simulink model "telescopio"  (R2025b)
settings: Solver=VariableStepAuto  StartTime=0.0  StopTime=15  RelTol=1e-3  AbsTol=1e-3
undefined symbols (not defined in the file): X, Y, Z
libraries: fl_lib x22, sm_lib x17, nesl_utility x17, ee_lib x6, slpidlib x3, simulink x3, sdl_lib x2
settings Model: Creator=kl247  LastModifiedBy=kl247
settings SolverCC: AutoScaleAbsTol=off  ZeroCrossAlgorithm=Adaptive  AlgebraicLoopSolver=TrustRegion  MaxZcPerStep=1.0
settings DebuggingCC: IgnoredZcDiagnostic=none  UnconnectedInputMsg=warning  UnconnectedOutputMsg=warning  UnconnectedLineMsg=warning  SymbolicDimsDataTypeCodeGenerationDiagnostic=none
settings ModelReferenceCC: EnableRefExpFcnMdlSchedulingChecks=on
settings SFSimCC: CustomCodeUndefinedFunction=UseInterfaceOnly
settings RTWCC: GPUComputeCapability=3.5  DLArmComputeVersion=19.05
settings SimscapeCC: SimscapeLogType=all  SimscapeLogSimulationStatistics=on  SimscapeLogDataHistory=10000.0

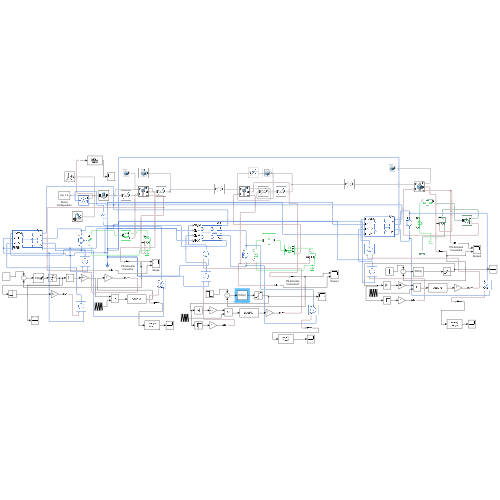
[thumbnail: Simulink's stored preview of the top-level diagram]
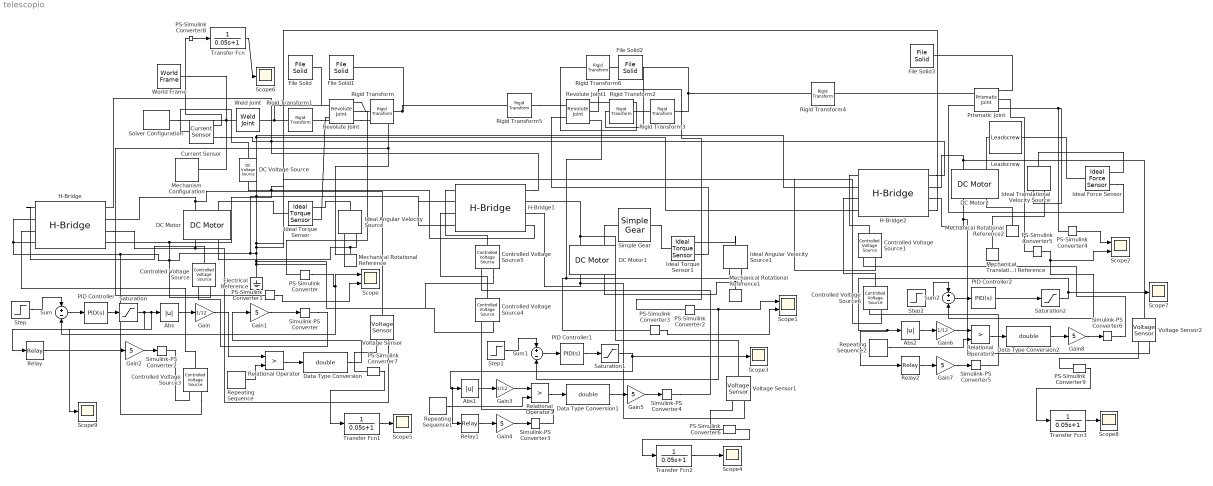
== system telescopio ==
  Abs : Abs  ZeroCross=off  SaturateOnIntegerOverflow=off
  Abs1 : Abs  ZeroCross=off  SaturateOnIntegerOverflow=off
  Abs2 : Abs  ZeroCross=off  SaturateOnIntegerOverflow=off
  Controlled Voltage Source{,1,3..6} (6 alike) : fl_lib/Electrical/Electrical Sources/Controlled Voltage Source
  Current Sensor : fl_lib/Electrical/Electrical Sensors/Current Sensor
  DC Motor : ee_lib/Electromechanical/Brushed Motors/DC Motor  field_option=ee.enum.field_option.pm  Rf=100 Ohm  Lf=1 H  Laf=0.15 H  If0=0 A  parameterization=ee.enum.dcparam_option.circuit_param  Ra=3.9 Ohm  La=12e-6 H  emf_or_torque=ee.enum.emf_or_torque.kv  Kv=0.072e-3 V/rpm  Ki=6.876e-4 N*m/A  T_stall=0.24e-3 N*m  w_max=19100 rpm  w_rated=15000 rpm  P_rated=0.08 W  V_rated=1.5 V  lam_param=ee.enum.lam_param.damping  i_noload=0 A  V_i_noload=1.5 V  J=0.01 cm^2*g  lam=0 N*m*s/rad  speed0=0 rpm  alpha=3.93e-3 1/K  Tmeas=25 degC  thermal_mass=100 J/K  initial_temperature=25 degC
  DC Motor1 : ee_lib/Electromechanical/Brushed Motors/DC Motor  field_option=ee.enum.field_option.pm  Rf=100 Ohm  Lf=1 H  Laf=0.15 H  If0=0 A  parameterization=ee.enum.dcparam_option.circuit_param  Ra=3.9 Ohm  La=12e-6 H  emf_or_torque=ee.enum.emf_or_torque.kv  Kv=0.072e-3 V/rpm  Ki=6.876e-4 N*m/A  T_stall=0.24e-3 N*m  w_max=19100 rpm  w_rated=15000 rpm  P_rated=0.08 W  V_rated=1.5 V  lam_param=ee.enum.lam_param.damping  i_noload=0 A  V_i_noload=1.5 V  J=0.01 cm^2*g  lam=0 N*m*s/rad  speed0=0 rpm  alpha=3.93e-3 1/K  Tmeas=25 degC  thermal_mass=100 J/K  initial_temperature=25 degC
  DC Motor2 : ee_lib/Electromechanical/Brushed Motors/DC Motor  field_option=ee.enum.field_option.pm  Rf=100 Ohm  Lf=1 H  Laf=0.15 H  If0=0 A  parameterization=ee.enum.dcparam_option.circuit_param  Ra=3.9 Ohm  La=12e-6 H  emf_or_torque=ee.enum.emf_or_torque.kv  Kv=0.072e-3 V/rpm  Ki=6.876e-4 N*m/A  T_stall=0.24e-3 N*m  w_max=19100 rpm  w_rated=15000 rpm  P_rated=0.08 W  V_rated=1.5 V  lam_param=ee.enum.lam_param.damping  i_noload=0 A  V_i_noload=1.5 V  J=0.01 cm^2*g  lam=0 N*m*s/rad  speed0=0 rpm  alpha=3.93e-3 1/K  Tmeas=25 degC  thermal_mass=100 J/K  initial_temperature=25 degC
  DC Voltage Source : fl_lib/Electrical/Electrical Sources/DC Voltage Source  v0=12 V
  Data Type Conversion : DataTypeConversion  OutDataTypeStr=double  SaturateOnIntegerOverflow=off  RndMeth=Floor
  Data Type Conversion1 : DataTypeConversion  OutDataTypeStr=double  SaturateOnIntegerOverflow=off  RndMeth=Floor
  Data Type Conversion2 : DataTypeConversion  OutDataTypeStr=double  SaturateOnIntegerOverflow=off  RndMeth=Floor
  Electrical Reference : fl_lib/Electrical/Electrical Elements/Electrical Reference
  File Solid : sm_lib/Body Elements/File Solid  ExtGeomFileName=C:\Users\kl247\OneDrive\Desktop\base_telescopio1.STEP  UnitType=FromFile  ExtGeomFileUnits=m  StepReaderType=HEX  ExportConvexHullGeometry=off  InertiaType=CalculateFromGeometry  BasedOnType=Density  Density=1200  DensityUnits=kg/m^3  Mass=1  MassUnits=kg  CenterOfMass=[0 0 0]  CenterOfMassUnits=m  MomentsOfInertia=[1 1 1]  MomentsOfInertiaUnits=kg*m^2  ProductsOfInertia=[0 0 0]  ProductsOfInertiaUnits=kg*m^2  GraphicType=FromGeometry  MarkerShape=Sphere  MarkerSize=10  GraphicVisPropType=SimpleVisualProperties  GraphicDiffuseColor=[0.5 0.5 0.5]  GraphicOpacity=1  GraphicSpecularColor=[0.5 0.5 0.5 1.0]  GraphicAmbientColor=[0.15 0.15 0.15 1.0]  GraphicEmissiveColor=[0.0 0.0 0.0 1.0]  GraphicShininess=75  DoExposeReferenceFrame=on  SerializedFrames=<Frames/>
  File Solid1 : sm_lib/Body Elements/File Solid  ExtGeomFileName=C:\Users\kl247\OneDrive\Desktop\soporte.STEP1.STEP  UnitType=FromFile  ExtGeomFileUnits=m  StepReaderType=HEX  ExportConvexHullGeometry=off  InertiaType=CalculateFromGeometry  BasedOnType=Density  Density=1200  DensityUnits=kg/m^3  Mass=1  MassUnits=kg  CenterOfMass=[0 0 0]  CenterOfMassUnits=m  MomentsOfInertia=[1 1 1]  MomentsOfInertiaUnits=kg*m^2  ProductsOfInertia=[0 0 0]  ProductsOfInertiaUnits=kg*m^2  GraphicType=FromGeometry  MarkerShape=Sphere  MarkerSize=10  GraphicVisPropType=SimpleVisualProperties  GraphicDiffuseColor=[0.5 0.5 0.5]  GraphicOpacity=1  GraphicSpecularColor=[0.5 0.5 0.5 1.0]  GraphicAmbientColor=[0.15 0.15 0.15 1.0]  GraphicEmissiveColor=[0.0 0.0 0.0 1.0]  GraphicShininess=75  DoExposeReferenceFrame=on  SerializedFrames=<Frames/>
  File Solid2 : sm_lib/Body Elements/File Solid  ExtGeomFileName=C:\Users\kl247\OneDrive\Desktop\tubo_exterior.STEP  UnitType=FromFile  ExtGeomFileUnits=m  StepReaderType=HEX  ExportConvexHullGeometry=off  InertiaType=CalculateFromGeometry  BasedOnType=Density  Density=300  DensityUnits=kg/m^3  Mass=1  MassUnits=kg  CenterOfMass=[0 0 0]  CenterOfMassUnits=m  MomentsOfInertia=[1 1 1]  MomentsOfInertiaUnits=kg*m^2  ProductsOfInertia=[0 0 0]  ProductsOfInertiaUnits=kg*m^2  GraphicType=FromGeometry  MarkerShape=Sphere  MarkerSize=10  GraphicVisPropType=SimpleVisualProperties  GraphicDiffuseColor=[0.5 0.5 0.5]  GraphicOpacity=1  GraphicSpecularColor=[0.5 0.5 0.5 1.0]  GraphicAmbientColor=[0.15 0.15 0.15 1.0]  GraphicEmissiveColor=[0.0 0.0 0.0 1.0]  GraphicShininess=75  DoExposeReferenceFrame=on  SerializedFrames=<Frames/>
  File Solid3 : sm_lib/Body Elements/File Solid  ExtGeomFileName=C:\Users\kl247\OneDrive\Desktop\tubo_interior.STEP  UnitType=FromFile  ExtGeomFileUnits=m  StepReaderType=HEX  ExportConvexHullGeometry=off  InertiaType=CalculateFromGeometry  BasedOnType=Density  Density=300  DensityUnits=kg/m^3  Mass=1  MassUnits=kg  CenterOfMass=[0 0 0]  CenterOfMassUnits=m  MomentsOfInertia=[1 1 1]  MomentsOfInertiaUnits=kg*m^2  ProductsOfInertia=[0 0 0]  ProductsOfInertiaUnits=kg*m^2  GraphicType=FromGeometry  MarkerShape=Sphere  MarkerSize=10  GraphicVisPropType=SimpleVisualProperties  GraphicDiffuseColor=[0.5 0.5 0.5]  GraphicOpacity=1  GraphicSpecularColor=[0.5 0.5 0.5 1.0]  GraphicAmbientColor=[0.15 0.15 0.15 1.0]  GraphicEmissiveColor=[0.0 0.0 0.0 1.0]  GraphicShininess=75  DoExposeReferenceFrame=on  SerializedFrames=<Frames/>
  Gain : Gain  Gain=1/12
  Gain{1..2,4..5,7..8} (6 alike) : Gain  Gain=5
  Gain3 : Gain  Gain=1/12
  Gain6 : Gain  Gain=1/12
  H-Bridge : ee_lib/Semiconductors & Converters/Converters/H-Bridge  supply_ports=ee.enum.supply_ports.showsupply  pwm_or_av=ee.enum.pwm_or_av.pwm  regenerative_braking_mode=ee.enum.converters.regenerative_braking_mode.depends_on_rev  discontinuous=ee.enum.current_profile.continuous  freewheeling_mode=ee.enum.converters.freewheeling_mode.one_switch_one_diode  Rload=10 Ohm  Lload=1e-5 H  F=10 kHz  Venable=2.5 V  Vmax=5.0 V  Vreverse=2.5 V  Vbrake=2.5 V  Vm=12 V  Ron=0.1 Ohm  Don=0.05 Ohm  Goff=1e-6 S  Tmeas=298.15 K  Ron2=0.1 Ohm  Don2=0.05 Ohm  Tmeas2=398.15 K  thermal_mass=100 J/K  initial_temperature=298.15 K
      settings: InternalSimscapePortConfiguration="{\"Bottom\":[],\"Left\":[{\"id\":\"ENA\",\"label\":\"PWM\",\"type\":\"foundation.electrical.electrical\"},{\"id\":\"REF\",\"label\":\"REF\",\"type\":\"foundation.electrical.electrical\"},{\"id\":\"REV\",\"label\":\"REV\",\"type\":\"foundation.electrical.electrical\"},{\"id\":\"BRK\",\"label\":\"BRK\",\"type\":\"foundation.electrical.electrical\"}],\"Right\":[{\"id\":\"p1\",\"label\":\"V+\",\"type\":\"foundation.electrical.electrical\"},{\"id\":\"p2\",\"label\":\"+\",\"type\":\"foundation.electrical.electrical\"},{\"id\":\"n2\",\"label\":\"-\",\"type\":\"foundation.electrical.electrical\"},{\"id\":\"n1\",\"label\":\"V-\",\"type\":\"foundation.electrical.electrical\"}],\"Top\":[]}"
  H-Bridge1 : ee_lib/Semiconductors & Converters/Converters/H-Bridge  supply_ports=ee.enum.supply_ports.showsupply  pwm_or_av=ee.enum.pwm_or_av.pwm  regenerative_braking_mode=ee.enum.converters.regenerative_braking_mode.depends_on_rev  discontinuous=ee.enum.current_profile.continuous  freewheeling_mode=ee.enum.converters.freewheeling_mode.one_switch_one_diode  Rload=10 Ohm  Lload=1e-5 H  F=10 kHz  Venable=2.5 V  Vmax=5.0 V  Vreverse=2.5 V  Vbrake=2.5 V  Vm=12 V  Ron=0.1 Ohm  Don=0.05 Ohm  Goff=1e-6 S  Tmeas=298.15 K  Ron2=0.1 Ohm  Don2=0.05 Ohm  Tmeas2=398.15 K  thermal_mass=100 J/K  initial_temperature=298.15 K
      settings: InternalSimscapePortConfiguration="{\"Bottom\":[],\"Left\":[{\"id\":\"ENA\",\"label\":\"PWM\",\"type\":\"foundation.electrical.electrical\"},{\"id\":\"REF\",\"label\":\"REF\",\"type\":\"foundation.electrical.electrical\"},{\"id\":\"REV\",\"label\":\"REV\",\"type\":\"foundation.electrical.electrical\"},{\"id\":\"BRK\",\"label\":\"BRK\",\"type\":\"foundation.electrical.electrical\"}],\"Right\":[{\"id\":\"p1\",\"label\":\"V+\",\"type\":\"foundation.electrical.electrical\"},{\"id\":\"p2\",\"label\":\"+\",\"type\":\"foundation.electrical.electrical\"},{\"id\":\"n2\",\"label\":\"-\",\"type\":\"foundation.electrical.electrical\"},{\"id\":\"n1\",\"label\":\"V-\",\"type\":\"foundation.electrical.electrical\"}],\"Top\":[]}"
  H-Bridge2 : ee_lib/Semiconductors & Converters/Converters/H-Bridge  supply_ports=ee.enum.supply_ports.showsupply  pwm_or_av=ee.enum.pwm_or_av.pwm  regenerative_braking_mode=ee.enum.converters.regenerative_braking_mode.depends_on_rev  discontinuous=ee.enum.current_profile.continuous  freewheeling_mode=ee.enum.converters.freewheeling_mode.one_switch_one_diode  Rload=10 Ohm  Lload=1e-5 H  F=10 kHz  Venable=2.5 V  Vmax=5.0 V  Vreverse=2.5 V  Vbrake=2.5 V  Vm=12 V  Ron=0.1 Ohm  Don=0.05 Ohm  Goff=1e-6 S  Tmeas=298.15 K  Ron2=0.1 Ohm  Don2=0.05 Ohm  Tmeas2=398.15 K  thermal_mass=100 J/K  initial_temperature=298.15 K
      settings: InternalSimscapePortConfiguration="{\"Bottom\":[],\"Left\":[{\"id\":\"ENA\",\"label\":\"PWM\",\"type\":\"foundation.electrical.electrical\"},{\"id\":\"REF\",\"label\":\"REF\",\"type\":\"foundation.electrical.electrical\"},{\"id\":\"REV\",\"label\":\"REV\",\"type\":\"foundation.electrical.electrical\"},{\"id\":\"BRK\",\"label\":\"BRK\",\"type\":\"foundation.electrical.electrical\"}],\"Right\":[{\"id\":\"p1\",\"label\":\"V+\",\"type\":\"foundation.electrical.electrical\"},{\"id\":\"p2\",\"label\":\"+\",\"type\":\"foundation.electrical.electrical\"},{\"id\":\"n2\",\"label\":\"-\",\"type\":\"foundation.electrical.electrical\"},{\"id\":\"n1\",\"label\":\"V-\",\"type\":\"foundation.electrical.electrical\"}],\"Top\":[]}"
  Ideal Angular Velocity Source : fl_lib/Mechanical/Mechanical Sources/Ideal Angular Velocity Source
  Ideal Angular Velocity Source1 : fl_lib/Mechanical/Mechanical Sources/Ideal Angular Velocity Source
  Ideal Force Sensor : fl_lib/Mechanical/Mechanical Sensors/Ideal Force Sensor
  Ideal Torque Sensor : fl_lib/Mechanical/Mechanical Sensors/Ideal Torque Sensor
  Ideal Torque Sensor1 : fl_lib/Mechanical/Mechanical Sensors/Ideal Torque Sensor
  Ideal Translational Velocity Source : fl_lib/Mechanical/Mechanical Sources/Ideal Translational Velocity Source
  Leadscrew : sdl_lib/Gears/Rotational- Translational/Leadscrew  Lead=0.015 m  helix_type=sdl.enum.handedness.right  friction_model=sdl.enum.gear_friction.none  friction_parameterization=sdl.enum.frictionParameterization.geometry  lambda=15 deg  alpha=14.5 deg  fr_coeff=0.08  eff_sn=0.75  eff_ns=0.45  temperature_TLU=[280, 300, 320] K  efficiency_sn_TLU=[.75, .65, .6]  efficiency_ns_TLU=[.5, .45, .4]  pwr_thr=0.001 W  mu_visc=0 N*m*s/rad  thermal_mass=50 J/K  temperature_specify=off  temperature_priority=High  temperature=300 K  temperature_nominal_specify=off  temperature_nominal_value=1  temperature_nominal_unit=K
      settings: InternalSimscapePortConfiguration="{\"Bottom\":[],\"Left\":[{\"id\":\"S\",\"label\":\"S\",\"type\":\"foundation.mechanical.rotational.rotational\"}],\"Right\":[{\"id\":\"N\",\"label\":\"N\",\"type\":\"foundation.mechanical.translational.translational\"}],\"Top\":[]}"
  Mechanical Rotational Reference : fl_lib/Mechanical/Rotational Elements/Mechanical Rotational Reference
  Mechanical Rotational Reference1 : fl_lib/Mechanical/Rotational Elements/Mechanical Rotational Reference
  Mechanical Rotational Reference2 : fl_lib/Mechanical/Rotational Elements/Mechanical Rotational Reference
  Mechanical Translational Reference : fl_lib/Mechanical/Translational Elements/Mechanical Translational Reference
  Mechanism Configuration : sm_lib/Utilities/Mechanism Configuration  UniformGravity=Constant  GravityVector=[0 0 -9.80665]  GravityVectorUnits=m/s^2  LinearizationDelta=0.001  JointModeTransitionNonlinearIterations=2
  PID Controller : slpidlib/PID Controller  Controller=PID  Form=Parallel  TimeDomain=Continuous-time  UseExternalTs=off  SampleTime=-1  IntegratorMethod=Forward Euler  FilterMethod=Forward Euler  ControllerParametersSource=internal  P=3  I=0  UseKiTs=off  D=10  UseExternalDerivativeSource=off  N=100  UseFilter=on  TunerSelectOption=Transfer Function Based (PID Tuner App)  InitialConditionSource=internal  InitialConditionForIntegrator=0  InitialConditionForFilter=0  DifferentiatorICPrevScaledInput=0  ExternalReset=none  TrackingMode=off  Kt=1  LimitOutput=on  SatLimitsSource=internal  UpperSaturationLimit=12  LowerSaturationLimit=-12  LinearizeAsGain=on  AntiWindupMode=none  Kb=1  LimitIntegrator=off  UpperIntegratorSaturationLimit=inf  LowerIntegratorSaturationLimit=-inf  POutMin=[]  POutMax=[]  IOutMin=[]  IOutMax=[]  DOutMin=[]  DOutMax=[]  NOutMin=[]  NOutMax=[]  SumOutMin=[]  SumOutMax=[]  SaturationOutMin=[]  SaturationOutMax=[]  PParamMin=[]  PParamMax=[]  IParamMin=[]  IParamMax=[]  DParamMin=[]  DParamMax=[]  NParamMin=[]  NParamMax=[]  KbParamMin=[]  KbParamMax=[]  KtParamMin=[]  KtParamMax=[]  KbOutMin=[]  KbOutMax=[]  KtOutMin=[]  KtOutMax=[]  IntegratorOutMin=[]  IntegratorOutMax=[]  FilterOutMin=[]  FilterOutMax=[]  SumI1OutMin=[]  SumI1OutMax=[]  SumI2OutMin=[]  SumI2OutMax=[]  SumI3OutMin=[]  SumI3OutMax=[]  SumI4OutMin=[]  SumI4OutMax=[]  SumDOutMin=[]  SumDOutMax=[]  DifferentiatorOutMin=[]  DifferentiatorOutMax=[]  FilterDiffOutCoefMin=[]  FilterDiffOutCoefMax=[]  ReciprocalOutMin=[]  ReciprocalOutMax=[]  SumDenOutMin=[]  SumDenOutMax=[]  SumNumOutMin=[]  SumNumOutMax=[]  DivideOutMin=[]  DivideOutMax=[]  UdiffTsProdOutMin=[]  UdiffTsProdOutMax=[]  NTsProdOutMin=[]  NTsProdOutMax=[]  UintegralTsProdOutMin=[]  UintegralTsProdOutMax=[]  UngainTsProdOutMin=[]  UngainTsProdOutMax=[]  ClampingZeroOutDataTypeStr=Inherit: Inherit via back propagation  ClampingZeroOutMin=[]  ClampingZeroOutMax=[]  FilterDenConstantOutDataTypeStr=Inherit: Inherit via back propagation  FilterDenConstantOutMin=[]  FilterDenConstantOutMax=[]  PCopyOutDataTypeStr=Inherit: Inherit via back propagation  PCopyOutMin=[]  PCopyOutMax=[]  NCopyOutDataTypeStr=Inherit: Inherit via back propagation  NCopyOutMin=[]  NCopyOutMax=[]  IntegratorContinuousStateAttributes=''  IntegratorStateMustResolveToSignalObject=off  IntegratorRTWStateStorageClass=Auto  FilterContinuousStateAttributes=''  FilterStateMustResolveToSignalObject=off  FilterRTWStateStorageClass=Auto  ParallelPVariant=InternalParameters  IdealPVariant=Disabled  IVariant=InternalParameters  DVariant=InternalParameters  IntegratorVariant=Continuous  SatVariant=Enabled  AWVariant=Passthrough  PCopyVariant=Disabled  TRVariant=Disabled  FdbkBlocksVariant=Forward  IdealPFdbkVariant=Disabled  SatFdbkVariant=Disabled  DerivativeFilterVariant=ContFilter  NVariant=InternalParameters  NCopyVariant=Disabled  FilterICVariant=InternalICsFilter  IntegratorICVariant=InternalICs  ExternalResetVariant=Disabled  TRSumVariant=Passthrough  SumFdbkVariant=Disabled  SumVariant=Sum_PID  TsampFilterVariant=InternalTs  TsampNgainVariant=Passthrough  TsampIntegralVariant=Disabled_SignalSpec  ExternalSaturationOutDataTypeStr=Inherit: Same as second input  DerivativeSourceVariant=ErrorSignal  PreIntVariant=InternalPreInt
  PID Controller1 : slpidlib/PID Controller  Controller=PID  Form=Parallel  TimeDomain=Continuous-time  UseExternalTs=off  SampleTime=-1  IntegratorMethod=Forward Euler  FilterMethod=Forward Euler  ControllerParametersSource=internal  P=30  I=2  UseKiTs=off  D=10  UseExternalDerivativeSource=off  N=100  UseFilter=on  TunerSelectOption=Transfer Function Based (PID Tuner App)  InitialConditionSource=internal  InitialConditionForIntegrator=0  InitialConditionForFilter=0  DifferentiatorICPrevScaledInput=0  ExternalReset=none  TrackingMode=off  Kt=1  LimitOutput=off  SatLimitsSource=internal  UpperSaturationLimit=inf  LowerSaturationLimit=-inf  LinearizeAsGain=on  AntiWindupMode=none  Kb=1  LimitIntegrator=off  UpperIntegratorSaturationLimit=inf  LowerIntegratorSaturationLimit=-inf  POutMin=[]  POutMax=[]  IOutMin=[]  IOutMax=[]  DOutMin=[]  DOutMax=[]  NOutMin=[]  NOutMax=[]  SumOutMin=[]  SumOutMax=[]  SaturationOutMin=[]  SaturationOutMax=[]  PParamMin=[]  PParamMax=[]  IParamMin=[]  IParamMax=[]  DParamMin=[]  DParamMax=[]  NParamMin=[]  NParamMax=[]  KbParamMin=[]  KbParamMax=[]  KtParamMin=[]  KtParamMax=[]  KbOutMin=[]  KbOutMax=[]  KtOutMin=[]  KtOutMax=[]  IntegratorOutMin=[]  IntegratorOutMax=[]  FilterOutMin=[]  FilterOutMax=[]  SumI1OutMin=[]  SumI1OutMax=[]  SumI2OutMin=[]  SumI2OutMax=[]  SumI3OutMin=[]  SumI3OutMax=[]  SumI4OutMin=[]  SumI4OutMax=[]  SumDOutMin=[]  SumDOutMax=[]  DifferentiatorOutMin=[]  DifferentiatorOutMax=[]  FilterDiffOutCoefMin=[]  FilterDiffOutCoefMax=[]  ReciprocalOutMin=[]  ReciprocalOutMax=[]  SumDenOutMin=[]  SumDenOutMax=[]  SumNumOutMin=[]  SumNumOutMax=[]  DivideOutMin=[]  DivideOutMax=[]  UdiffTsProdOutMin=[]  UdiffTsProdOutMax=[]  NTsProdOutMin=[]  NTsProdOutMax=[]  UintegralTsProdOutMin=[]  UintegralTsProdOutMax=[]  UngainTsProdOutMin=[]  UngainTsProdOutMax=[]  ClampingZeroOutDataTypeStr=Inherit: Inherit via back propagation  ClampingZeroOutMin=[]  ClampingZeroOutMax=[]  FilterDenConstantOutDataTypeStr=Inherit: Inherit via back propagation  FilterDenConstantOutMin=[]  FilterDenConstantOutMax=[]  PCopyOutDataTypeStr=Inherit: Inherit via back propagation  PCopyOutMin=[]  PCopyOutMax=[]  NCopyOutDataTypeStr=Inherit: Inherit via back propagation  NCopyOutMin=[]  NCopyOutMax=[]  IntegratorContinuousStateAttributes=''  IntegratorStateMustResolveToSignalObject=off  IntegratorRTWStateStorageClass=Auto  FilterContinuousStateAttributes=''  FilterStateMustResolveToSignalObject=off  FilterRTWStateStorageClass=Auto  ParallelPVariant=InternalParameters  IdealPVariant=Disabled  IVariant=InternalParameters  DVariant=InternalParameters  IntegratorVariant=Continuous  SatVariant=Disabled  AWVariant=Passthrough  PCopyVariant=Disabled  TRVariant=Disabled  FdbkBlocksVariant=Forward  IdealPFdbkVariant=Disabled  SatFdbkVariant=Disabled  DerivativeFilterVariant=ContFilter  NVariant=InternalParameters  NCopyVariant=Disabled  FilterICVariant=InternalICsFilter  IntegratorICVariant=InternalICs  ExternalResetVariant=Disabled  TRSumVariant=Passthrough  SumFdbkVariant=Disabled  SumVariant=Sum_PID  TsampFilterVariant=InternalTs  TsampNgainVariant=Passthrough  TsampIntegralVariant=Disabled_SignalSpec  ExternalSaturationOutDataTypeStr=Inherit: Same as second input  DerivativeSourceVariant=ErrorSignal  PreIntVariant=InternalPreInt
  PID Controller2 : slpidlib/PID Controller  Controller=PID  Form=Parallel  TimeDomain=Continuous-time  UseExternalTs=off  SampleTime=-1  IntegratorMethod=Forward Euler  FilterMethod=Forward Euler  ControllerParametersSource=internal  P=500  I=0  UseKiTs=off  D=0  UseExternalDerivativeSource=off  N=100  UseFilter=on  TunerSelectOption=Transfer Function Based (PID Tuner App)  InitialConditionSource=internal  InitialConditionForIntegrator=0  InitialConditionForFilter=0  DifferentiatorICPrevScaledInput=0  ExternalReset=none  TrackingMode=off  Kt=1  LimitOutput=off  SatLimitsSource=internal  UpperSaturationLimit=inf  LowerSaturationLimit=-inf  LinearizeAsGain=on  AntiWindupMode=none  Kb=1  LimitIntegrator=off  UpperIntegratorSaturationLimit=inf  LowerIntegratorSaturationLimit=-inf  POutMin=[]  POutMax=[]  IOutMin=[]  IOutMax=[]  DOutMin=[]  DOutMax=[]  NOutMin=[]  NOutMax=[]  SumOutMin=[]  SumOutMax=[]  SaturationOutMin=[]  SaturationOutMax=[]  PParamMin=[]  PParamMax=[]  IParamMin=[]  IParamMax=[]  DParamMin=[]  DParamMax=[]  NParamMin=[]  NParamMax=[]  KbParamMin=[]  KbParamMax=[]  KtParamMin=[]  KtParamMax=[]  KbOutMin=[]  KbOutMax=[]  KtOutMin=[]  KtOutMax=[]  IntegratorOutMin=[]  IntegratorOutMax=[]  FilterOutMin=[]  FilterOutMax=[]  SumI1OutMin=[]  SumI1OutMax=[]  SumI2OutMin=[]  SumI2OutMax=[]  SumI3OutMin=[]  SumI3OutMax=[]  SumI4OutMin=[]  SumI4OutMax=[]  SumDOutMin=[]  SumDOutMax=[]  DifferentiatorOutMin=[]  DifferentiatorOutMax=[]  FilterDiffOutCoefMin=[]  FilterDiffOutCoefMax=[]  ReciprocalOutMin=[]  ReciprocalOutMax=[]  SumDenOutMin=[]  SumDenOutMax=[]  SumNumOutMin=[]  SumNumOutMax=[]  DivideOutMin=[]  DivideOutMax=[]  UdiffTsProdOutMin=[]  UdiffTsProdOutMax=[]  NTsProdOutMin=[]  NTsProdOutMax=[]  UintegralTsProdOutMin=[]  UintegralTsProdOutMax=[]  UngainTsProdOutMin=[]  UngainTsProdOutMax=[]  ClampingZeroOutDataTypeStr=Inherit: Inherit via back propagation  ClampingZeroOutMin=[]  ClampingZeroOutMax=[]  FilterDenConstantOutDataTypeStr=Inherit: Inherit via back propagation  FilterDenConstantOutMin=[]  FilterDenConstantOutMax=[]  PCopyOutDataTypeStr=Inherit: Inherit via back propagation  PCopyOutMin=[]  PCopyOutMax=[]  NCopyOutDataTypeStr=Inherit: Inherit via back propagation  NCopyOutMin=[]  NCopyOutMax=[]  IntegratorContinuousStateAttributes=''  IntegratorStateMustResolveToSignalObject=off  IntegratorRTWStateStorageClass=Auto  FilterContinuousStateAttributes=''  FilterStateMustResolveToSignalObject=off  FilterRTWStateStorageClass=Auto  ParallelPVariant=InternalParameters  IdealPVariant=Disabled  IVariant=InternalParameters  DVariant=InternalParameters  IntegratorVariant=Continuous  SatVariant=Disabled  AWVariant=Passthrough  PCopyVariant=Disabled  TRVariant=Disabled  FdbkBlocksVariant=Forward  IdealPFdbkVariant=Disabled  SatFdbkVariant=Disabled  DerivativeFilterVariant=ContFilter  NVariant=InternalParameters  NCopyVariant=Disabled  FilterICVariant=InternalICsFilter  IntegratorICVariant=InternalICs  ExternalResetVariant=Disabled  TRSumVariant=Passthrough  SumFdbkVariant=Disabled  SumVariant=Sum_PID  TsampFilterVariant=InternalTs  TsampNgainVariant=Passthrough  TsampIntegralVariant=Disabled_SignalSpec  ExternalSaturationOutDataTypeStr=Inherit: Same as second input  DerivativeSourceVariant=ErrorSignal  PreIntVariant=InternalPreInt
  PS-Simulink Converter{,1..9} (10 alike) : nesl_utility/PS-Simulink Converter  PhysicalDomain=network_engine_domain  SubClassName=ps_output  LeftPortType=input  RightPortType=output  PseudoPeriodic=off  Frequencies=[]  VectorFormat=inherit  Unit=inherit  AffineConversion=off
  Prismatic Joint : sm_lib/Joints/Prismatic Joint  JointMode=Normal  CompositeWrenchDir=FollowerOnBase  CompositeWrenchFrame=BaseFrame  SenseConstraintForce=off  SenseConstraintTorque=off  SenseTotalForce=off  SenseTotalTorque=off  PositionTargetSpecify=off  PositionTargetPriority=High  PositionTargetValue=0  PositionTargetValueUnits=m  VelocityTargetSpecify=off  VelocityTargetPriority=High  VelocityTargetValue=0  VelocityTargetValueUnits=m/s  EquilibriumPosition=0  EquilibriumPositionUnits=m  SpringStiffness=0  SpringStiffnessUnits=N/m  DampingCoefficient=50  DampingCoefficientUnits=N/(m/s)  LowerLimitSpecify=off  LowerLimitBound=-1  LowerLimitBoundUnits=m  LowerLimitStiffness=1e6  LowerLimitStiffnessUnits=N/m  LowerLimitDamping=1e3  LowerLimitDampingUnits=N/(m/s)  LowerLimitTransitionRegionWidth=1e-4  LowerLimitTransitionRegionWidthUnits=m  UpperLimitSpecify=off  UpperLimitBound=1  UpperLimitBoundUnits=m  UpperLimitStiffness=1e6  UpperLimitStiffnessUnits=N/m  UpperLimitDamping=1e3  UpperLimitDampingUnits=N/(m/s)  UpperLimitTransitionRegionWidth=1e-4  UpperLimitTransitionRegionWidthUnits=m  TorqueActuationMode=InputTorque  MotionActuationMode=ComputedMotion  SensePosition=on  SenseVelocity=on  SenseAcceleration=off  SenseTorqueForce=off  SenseLowerLimitTorqueForce=off  SenseUpperLimitTorqueForce=off
  Relational Operator : RelationalOperator  Operator=>  OutDataTypeStr=boolean  RndMeth=Simplest  InputSameDT=off
  Relational Operator1 : RelationalOperator  Operator=>  OutDataTypeStr=boolean  RndMeth=Simplest  InputSameDT=off
  Relational Operator2 : RelationalOperator  Operator=>  OutDataTypeStr=boolean  RndMeth=Simplest  InputSameDT=off
  Relay : Relay  OnSwitchValue=0.5  OffSwitchValue=-0.5  OnOutputValue=0  OffOutputValue=1
  Relay1 : Relay  OnSwitchValue=0.5  OffSwitchValue=-0.5  OnOutputValue=0  OffOutputValue=1
  Relay2 : Relay  OnSwitchValue=0.5  OffSwitchValue=-0.5  OnOutputValue=0  OffOutputValue=1
  Repeating Sequence : simulink/Sources/Repeating Sequence  rep_seq_t=[0 0.001 0.002]  rep_seq_y=[0.01 0.99 0.01]
  Repeating Sequence1 : simulink/Sources/Repeating Sequence  rep_seq_t=[0 0.001 0.002]  rep_seq_y=[0.01 0.99 0.01]
  Repeating Sequence2 : simulink/Sources/Repeating Sequence  rep_seq_t=[0 0.001 0.002]  rep_seq_y=[0.01 0.99 0.01]
  Revolute Joint : sm_lib/Joints/Revolute Joint  JointMode=Normal  CompositeWrenchDir=FollowerOnBase  CompositeWrenchFrame=BaseFrame  SenseConstraintForce=off  SenseConstraintTorque=off  SenseTotalForce=off  SenseTotalTorque=off  PositionTargetSpecify=off  PositionTargetPriority=High  PositionTargetValue=0  PositionTargetValueUnits=deg  VelocityTargetSpecify=off  VelocityTargetPriority=High  VelocityTargetValue=0  VelocityTargetValueUnits=deg/s  EquilibriumPosition=0  EquilibriumPositionUnits=deg  SpringStiffness=0  SpringStiffnessUnits=N*m/deg  DampingCoefficient=0  DampingCoefficientUnits=N*m/(deg/s)  LowerLimitSpecify=off  LowerLimitBound=-90  LowerLimitBoundUnits=deg  LowerLimitStiffness=1e4  LowerLimitStiffnessUnits=N*m/deg  LowerLimitDamping=10  LowerLimitDampingUnits=N*m/(deg/s)  LowerLimitTransitionRegionWidth=0.1  LowerLimitTransitionRegionWidthUnits=deg  UpperLimitSpecify=off  UpperLimitBound=90  UpperLimitBoundUnits=deg  UpperLimitStiffness=1e4  UpperLimitStiffnessUnits=N*m/deg  UpperLimitDamping=10  UpperLimitDampingUnits=N*m/(deg/s)  UpperLimitTransitionRegionWidth=0.1  UpperLimitTransitionRegionWidthUnits=deg  TorqueActuationMode=InputTorque  MotionActuationMode=ComputedMotion  SensePosition=on  SenseVelocity=on  SenseAcceleration=off  SenseTorqueForce=off  SenseLowerLimitTorqueForce=off  SenseUpperLimitTorqueForce=off
  Revolute Joint1 : sm_lib/Joints/Revolute Joint  JointMode=Normal  CompositeWrenchDir=FollowerOnBase  CompositeWrenchFrame=BaseFrame  SenseConstraintForce=off  SenseConstraintTorque=off  SenseTotalForce=off  SenseTotalTorque=off  PositionTargetSpecify=off  PositionTargetPriority=High  PositionTargetValue=0  PositionTargetValueUnits=deg  VelocityTargetSpecify=off  VelocityTargetPriority=High  VelocityTargetValue=0  VelocityTargetValueUnits=deg/s  EquilibriumPosition=0  EquilibriumPositionUnits=deg  SpringStiffness=0  SpringStiffnessUnits=N*m/deg  DampingCoefficient=0.01  DampingCoefficientUnits=N*m/(deg/s)  LowerLimitSpecify=off  LowerLimitBound=-90  LowerLimitBoundUnits=deg  LowerLimitStiffness=1e4  LowerLimitStiffnessUnits=N*m/deg  LowerLimitDamping=10  LowerLimitDampingUnits=N*m/(deg/s)  LowerLimitTransitionRegionWidth=0.1  LowerLimitTransitionRegionWidthUnits=deg  UpperLimitSpecify=off  UpperLimitBound=90  UpperLimitBoundUnits=deg  UpperLimitStiffness=1e4  UpperLimitStiffnessUnits=N*m/deg  UpperLimitDamping=10  UpperLimitDampingUnits=N*m/(deg/s)  UpperLimitTransitionRegionWidth=0.1  UpperLimitTransitionRegionWidthUnits=deg  TorqueActuationMode=InputTorque  MotionActuationMode=ComputedMotion  SensePosition=on  SenseVelocity=on  SenseAcceleration=off  SenseTorqueForce=off  SenseLowerLimitTorqueForce=off  SenseUpperLimitTorqueForce=off
  Rigid Transform : sm_lib/Frames and Transforms/Rigid Transform  RotationMethod=StandardAxis  FollAlignAxisA=+X  BaseAlignAxisA=+Y  FollAlignAxisB=+Y  BaseAlignAxisB=+Z  RotationStandardAxis=+X  RotationAngle=90  RotationAngleUnits=deg  RotationArbitraryAxis=[0 0 1]  RotationSequenceAxes=FollowerAxes  RotationSequence=XYX  RotationSequenceAngles=[0 0 0]  RotationSequenceAnglesUnits=deg  RotationMatrix=[1 0 0;0 1 0;0 0 1]  Quaternion=[1 0 0 0]  TranslationMethod=Cartesian  TranslationCartesianOffset=[0 0 68]  TranslationCartesianOffsetUnits=mm  TranslationStandardAxis=+Z  TranslationStandardOffset=0  TranslationStandardOffsetUnits=m  TranslationROffset=0  TranslationROffsetUnits=m  TranslationThetaOffset=0  TranslationThetaOffsetUnits=deg  TranslationZOffset=0  TranslationZOffsetUnits=m
  Rigid Transform1 : sm_lib/Frames and Transforms/Rigid Transform  RotationMethod=StandardAxis  FollAlignAxisA=+X  BaseAlignAxisA=+Y  FollAlignAxisB=+Y  BaseAlignAxisB=+Z  RotationStandardAxis=+X  RotationAngle=90  RotationAngleUnits=deg  RotationArbitraryAxis=[0 0 1]  RotationSequenceAxes=FollowerAxes  RotationSequence=XYX  RotationSequenceAngles=[0 0 0]  RotationSequenceAnglesUnits=deg  RotationMatrix=[1 0 0;0 1 0;0 0 1]  Quaternion=[1 0 0 0]  TranslationMethod=None  TranslationCartesianOffset=[0 0 0]  TranslationCartesianOffsetUnits=m  TranslationStandardAxis=+Z  TranslationStandardOffset=0  TranslationStandardOffsetUnits=m  TranslationROffset=0  TranslationROffsetUnits=m  TranslationThetaOffset=0  TranslationThetaOffsetUnits=deg  TranslationZOffset=0  TranslationZOffsetUnits=m
  Rigid Transform2 : sm_lib/Frames and Transforms/Rigid Transform  RotationMethod=StandardAxis  FollAlignAxisA=+X  BaseAlignAxisA=+Y  FollAlignAxisB=+Y  BaseAlignAxisB=+Z  RotationStandardAxis=-X  RotationAngle=90  RotationAngleUnits=deg  RotationArbitraryAxis=[0 0 1]  RotationSequenceAxes=FollowerAxes  RotationSequence=XYX  RotationSequenceAngles=[0 0 0]  RotationSequenceAnglesUnits=deg  RotationMatrix=[1 0 0;0 1 0;0 0 1]  Quaternion=[1 0 0 0]  TranslationMethod=Cartesian  TranslationCartesianOffset=[0 0 0]  TranslationCartesianOffsetUnits=mm  TranslationStandardAxis=+Z  TranslationStandardOffset=0  TranslationStandardOffsetUnits=m  TranslationROffset=0  TranslationROffsetUnits=m  TranslationThetaOffset=0  TranslationThetaOffsetUnits=deg  TranslationZOffset=0  TranslationZOffsetUnits=m
  Rigid Transform3 : sm_lib/Frames and Transforms/Rigid Transform  RotationMethod=StandardAxis  FollAlignAxisA=+X  BaseAlignAxisA=+Y  FollAlignAxisB=+Y  BaseAlignAxisB=+Z  RotationStandardAxis=-Y  RotationAngle=90  RotationAngleUnits=deg  RotationArbitraryAxis=[0 0 1]  RotationSequenceAxes=FollowerAxes  RotationSequence=XYX  RotationSequenceAngles=[0 0 0]  RotationSequenceAnglesUnits=deg  RotationMatrix=[1 0 0;0 1 0;0 0 1]  Quaternion=[1 0 0 0]  TranslationMethod=None  TranslationCartesianOffset=[0 0 0]  TranslationCartesianOffsetUnits=m  TranslationStandardAxis=+Z  TranslationStandardOffset=0  TranslationStandardOffsetUnits=m  TranslationROffset=0  TranslationROffsetUnits=m  TranslationThetaOffset=0  TranslationThetaOffsetUnits=deg  TranslationZOffset=0  TranslationZOffsetUnits=m
  Rigid Transform4 : sm_lib/Frames and Transforms/Rigid Transform  RotationMethod=StandardAxis  FollAlignAxisA=+X  BaseAlignAxisA=+Y  FollAlignAxisB=+Y  BaseAlignAxisB=+Z  RotationStandardAxis=-X  RotationAngle=90  RotationAngleUnits=deg  RotationArbitraryAxis=[0 0 1]  RotationSequenceAxes=FollowerAxes  RotationSequence=XYX  RotationSequenceAngles=[0 0 0]  RotationSequenceAnglesUnits=deg  RotationMatrix=[1 0 0;0 1 0;0 0 1]  Quaternion=[1 0 0 0]  TranslationMethod=Cartesian  TranslationCartesianOffset=[0 0 0]  TranslationCartesianOffsetUnits=mm  TranslationStandardAxis=+Z  TranslationStandardOffset=0  TranslationStandardOffsetUnits=m  TranslationROffset=0  TranslationROffsetUnits=m  TranslationThetaOffset=0  TranslationThetaOffsetUnits=deg  TranslationZOffset=0  TranslationZOffsetUnits=m
  Rigid Transform5 : sm_lib/Frames and Transforms/Rigid Transform  RotationMethod=StandardAxis  FollAlignAxisA=+X  BaseAlignAxisA=+Y  FollAlignAxisB=+Y  BaseAlignAxisB=+Z  RotationStandardAxis=+Y  RotationAngle=90  RotationAngleUnits=deg  RotationArbitraryAxis=[0 0 1]  RotationSequenceAxes=FollowerAxes  RotationSequence=XYX  RotationSequenceAngles=[0 0 0]  RotationSequenceAnglesUnits=deg  RotationMatrix=[1 0 0;0 1 0;0 0 1]  Quaternion=[1 0 0 0]  TranslationMethod=Cartesian  TranslationCartesianOffset=[0 98 0]  TranslationCartesianOffsetUnits=mm  TranslationStandardAxis=+Z  TranslationStandardOffset=0  TranslationStandardOffsetUnits=m  TranslationROffset=0  TranslationROffsetUnits=m  TranslationThetaOffset=0  TranslationThetaOffsetUnits=deg  TranslationZOffset=0  TranslationZOffsetUnits=m
  Rigid Transform6 : sm_lib/Frames and Transforms/Rigid Transform  RotationMethod=StandardAxis  FollAlignAxisA=+X  BaseAlignAxisA=+Y  FollAlignAxisB=+Y  BaseAlignAxisB=+Z  RotationStandardAxis=-Y  RotationAngle=90  RotationAngleUnits=deg  RotationArbitraryAxis=[0 0 1]  RotationSequenceAxes=FollowerAxes  RotationSequence=XYX  RotationSequenceAngles=[0 0 0]  RotationSequenceAnglesUnits=deg  RotationMatrix=[1 0 0;0 1 0;0 0 1]  Quaternion=[1 0 0 0]  TranslationMethod=None  TranslationCartesianOffset=[0 0 0]  TranslationCartesianOffsetUnits=m  TranslationStandardAxis=+Z  TranslationStandardOffset=0  TranslationStandardOffsetUnits=m  TranslationROffset=0  TranslationROffsetUnits=m  TranslationThetaOffset=0  TranslationThetaOffsetUnits=deg  TranslationZOffset=0  TranslationZOffsetUnits=m
  Saturation : Saturate  UpperLimit=12  LowerLimit=-12
  Saturation1 : Saturate  UpperLimit=12  LowerLimit=-12
  Saturation2 : Saturate  UpperLimit=12  LowerLimit=-12
  Scope : Scope  NumInputPorts=2
      settings: ActiveDisplayYMinimum=-1  ActiveDisplayYMaximum=1
  Scope1 : Scope  NumInputPorts=2
      settings: ActiveDisplayYMinimum=-1  ActiveDisplayYMaximum=1
  Scope2 : Scope  NumInputPorts=2
      settings: ActiveDisplayYMinimum=-0.13293207584373259  ActiveDisplayYMaximum=0.12685054648463642  DataLoggingVariableName=ScopeData2
  Scope{3..9} (7 alike) : Scope
      Scope3 settings: ActiveDisplayYMinimum=-1  ActiveDisplayYMaximum=1  DataLoggingVariableName=ScopeData3
      Scope4 settings: ActiveDisplayYMinimum=-8.6927503970823583  ActiveDisplayYMaximum=1.4729668615940592  DataLoggingVariableName=ScopeData4
      Scope5 settings: ActiveDisplayYMinimum=-1.598657312003976  ActiveDisplayYMaximum=8.4258222495527821  DataLoggingVariableName=ScopeData5
      Scope6 settings: ActiveDisplayYMinimum=-1  ActiveDisplayYMaximum=1  DataLoggingVariableName=ScopeData6
      Scope7 settings: ActiveDisplayYMinimum=-13.50000000899878  ActiveDisplayYMaximum=1.5000000809890306  DataLoggingVariableName=ScopeData7
      Scope8 settings: ActiveDisplayYMinimum=-13.162620198868545  ActiveDisplayYMaximum=1.4625133554298382  DataLoggingVariableName=ScopeData8
      Scope9 settings: ActiveDisplayYMinimum=-2.0914538993512273  ActiveDisplayYMaximum=13.565717099927914  DataLoggingVariableName=ScopeData9
  Simple Gear : sdl_lib/Gears/Simple Gear  ratio=200  rotation_direction=sdl.enum.shaftOutputDirection.same  friction_model=sdl.enum.gear_efficiencies_load.off  T_noload=0.1 N*m  T_nom=5 N*m  efficiency_nom=0.8  efficiency=0.8  temperature_TLU=[280, 300, 320] K  load_TLU=[1, 5, 10] N*m  efficiency_TLU=[.95, .9, .85]  efficiency_TLU2=[.85, .8, .75; .95, .9, .85; .85, .8, .7]  w_thr=0.01 rad/s  pwr_thr=0.001 W  enable_backlash=false  hardstop_model=simscape.enum.hardstop.smooth  backlash_distance=1e-3 mm  r_base=0.1 m  transition=1e-4 mm  backlash_stiffness=1e6 N/m  backlash_damping=1e3 N*s/m  coeff_rest=0.7  v_tol=0.001 m/s  f_tol=0.001 N  mu_visc=[0, 0] N*m*s/rad  thermal_mass=50 J/K  temperature_specify=off  temperature_priority=High  temperature=300 K  temperature_nominal_specify=off  temperature_nominal_value=1  temperature_nominal_unit=K  x_backlash_specify=off  x_backlash_priority=None  x_backlash=0 mm  x_backlash_nominal_specify=off  x_backlash_nominal_value=1  x_backlash_nominal_unit=mm  f_hardstop_specify=off  f_hardstop_priority=None  f_hardstop=0 N  f_hardstop_nominal_specify=off  f_hardstop_nominal_value=1  f_hardstop_nominal_unit=N  v_backlash_specify=off  v_backlash_priority=None  v_backlash=0 m/s  v_backlash_nominal_specify=off  v_backlash_nominal_value=1  v_backlash_nominal_unit=m/s
  Simulink-PS Converter{,2..6} (6 alike) : nesl_utility/Simulink-PS Converter  PhysicalDomain=network_engine_domain  SubClassName=ps_input  LeftPortType=input  RightPortType=output  PseudoPeriodic=off  Frequencies=[]  NoiseDistribution=none  NoiseParameters=[]  Unit=1  AffineConversion=off  FilteringAndDerivatives=provide  SimscapeFilterOrder=1  InputFilterTimeConstant=0.001  UdotUserProvided=0
  Solver Configuration : nesl_utility/Solver Configuration  PhysicalDomain=network_engine_domain  SubClassName=solver  LeftPortType=input  RightPortType=generic  Tones=[]  Harmonics=[]  SimulateNoise=off  Profile=off  UseLocalSampling=off  EnableSwitchedLinearOptims=on  FrequencyDomain=off  UseCCode=off  RelTol=0.001  AbsTol=1e-06  MinStep=1e-09  ToWorkspace=off  RevertToSquareIcSolve=off  NumHomotopyIterations=100  PhasorMode=off  PhasorModeNumHarmonics=1  ConsistencySolver=NEWTON_XTOL_AFTER_FTOL  IndexReductionMethod=DerivativeReplacement  DoDC=off  ResidualTolerance=1e-09  ConsistencyTolSource=GLOBAL  ConsistencyAbsTol=0.001  ConsistencyRelTol=0.001  ConsistencyTolFactor=0.001  UseLocalSolver=on  LocalSolverChoice=NE_BACKWARD_EULER_ADVANCER  ResolveIndetEquations=on  FunctionEvalNumThread=1  LocalSolverSampleTime=1e-4  DoFixedCost=off  MaxNonlinIter=3  MaxModeIter=2  ComputeImpulses=off  ImpulseIterations=2  LinearAlgebra=auto  LinearAlgebraNumThread=0  EquationFormulation=NE_TIME_EF  DelaysMemoryBudget=1024  AutomaticFiltering=on  FilteringTimeConstant=0.001  PartitionStorageMethod=AS_NEEDED  PartitionMemoryBudget=1024  PartitionMethod=ROBUST  MultibodyUseLocalSolver=off  MultibodyLocalSolverChoice=ODE1  MultibodyLocalSolverSampleTime=0.001
  Step : Step  SampleTime=0
  Step1 : Step  After=-0.5  SampleTime=0
  Step2 : Step  After=-0.12  SampleTime=0
  Sum : Sum  Inputs=+-
  Sum1 : Sum  Inputs=+-
  Sum2 : Sum  Inputs=+-
  Transfer Fcn{,1..3} (4 alike) : TransferFcn  Denominator=[0.05 1]
  Voltage Sensor : fl_lib/Electrical/Electrical Sensors/Voltage Sensor
  Voltage Sensor1 : fl_lib/Electrical/Electrical Sensors/Voltage Sensor
  Voltage Sensor2 : fl_lib/Electrical/Electrical Sensors/Voltage Sensor
  Weld Joint : sm_lib/Joints/Weld Joint  JointMode=Normal  CompositeWrenchDir=FollowerOnBase  CompositeWrenchFrame=BaseFrame  SenseConstraintForce=off  SenseConstraintTorque=off  SenseTotalForce=off  SenseTotalTorque=off
  World Frame : sm_lib/Frames and Transforms/World Frame
  wires:
  PS-Simulink Converter/1 -> Sum/2, Scope/1
  PS-Simulink Converter1/1 -> Scope/2
  Step/1 -> Sum/1
  Sum/1 -> PID Controller/1
  PID Controller/1 -> Saturation/1
  Sum1/1 -> PID Controller1/1
  PID Controller1/1 -> Saturation1/1
  Step1/1 -> Sum1/1
  PS-Simulink Converter3/1 -> Scope1/2
  PS-Simulink Converter2/1 -> Sum1/2, Scope1/1
  PS-Simulink Converter5/1 -> Sum2/2, Scope2/2
  PS-Simulink Converter4/1 -> Scope2/1
  Step2/1 -> Sum2/1
  Sum2/1 -> PID Controller2/1
  PID Controller2/1 -> Saturation2/1
  Saturation/1 -> Scope9/1, Relay/1, Abs/1
  Abs/1 -> Gain/1
  Relay/1 -> Gain2/1
  Gain2/1 -> Simulink-PS Converter2/1
  Gain1/1 -> Simulink-PS Converter/1
  Gain/1 -> Relational Operator/1
  Repeating Sequence/1 -> Relational Operator/2
  Relational Operator/1 -> Data Type Conversion/1
  Data Type Conversion/1 -> Gain1/1
  Abs1/1 -> Gain3/1
  Gain3/1 -> Relational Operator1/1
  Relational Operator1/1 -> Data Type Conversion1/1
  Data Type Conversion1/1 -> Gain5/1
  Gain5/1 -> Simulink-PS Converter4/1
  Relay1/1 -> Gain4/1
  Gain4/1 -> Simulink-PS Converter3/1
  Repeating Sequence1/1 -> Relational Operator1/2
  Saturation1/1 -> Relay1/1, Abs1/1, Scope3/1
  Relational Operator2/1 -> Data Type Conversion2/1
  Abs2/1 -> Gain6/1
  Data Type Conversion2/1 -> Gain8/1
  Gain8/1 -> Simulink-PS Converter6/1
  Repeating Sequence2/1 -> Relational Operator2/2
  Gain6/1 -> Relational Operator2/1
  Gain7/1 -> Simulink-PS Converter5/1
  Relay2/1 -> Gain7/1
  Saturation2/1 -> Scope7/1, Relay2/1, Abs2/1
  PS-Simulink Converter8/1 -> Transfer Fcn/1
  Transfer Fcn/1 -> Scope6/1
  PS-Simulink Converter7/1 -> Transfer Fcn1/1
  Transfer Fcn1/1 -> Scope5/1
  Transfer Fcn2/1 -> Scope4/1
  PS-Simulink Converter6/1 -> Transfer Fcn2/1
  Transfer Fcn3/1 -> Scope8/1
  PS-Simulink Converter9/1 -> Transfer Fcn3/1
  connections:
  World Frame/RConn1 -- Mechanism Configuration/RConn1 -- Weld Joint/LConn1 -- Solver Configuration/RConn1
  Rigid Transform1/RConn1 -- File Solid/RConn1
  Revolute Joint/RConn1 -- Rigid Transform/LConn1
  Rigid Transform/RConn1 -- File Solid1/RConn1 -- Rigid Transform5/LConn1
  Rigid Transform1/LConn1 -- Revolute Joint/LConn1 -- Weld Joint/RConn1
  Rigid Transform3/LConn1 -- Rigid Transform2/RConn1
  Rigid Transform3/RConn1 -- Rigid Transform4/LConn1 -- File Solid2/RConn1
  Ideal Angular Velocity Source/RConn2 -- DC Motor/RConn2 -- Mechanical Rotational Reference/LConn1
  Ideal Angular Velocity Source/LConn1 -- Ideal Torque Sensor/RConn1
  Revolute Joint/RConn3 -- PS-Simulink Converter1/LConn1 -- Ideal Angular Velocity Source/RConn1
  Ideal Torque Sensor/RConn2 -- Revolute Joint/LConn2
  DC Motor/LConn2 -- Ideal Torque Sensor/LConn1
  Electrical Reference/LConn1 -- Controlled Voltage Source6/RConn2 -- Controlled Voltage Source1/RConn2 -- H-Bridge2/LConn4 -- H-Bridge2/LConn2 -- H-Bridge1/LConn4 -- H-Bridge1/LConn2 -- H-Bridge/LConn4 -- H-Bridge/LConn2 -- Controlled Voltage Source3/RConn2 -- H-Bridge1/RConn4 -- H-Bridge2/RConn4 -- DC Voltage Source/RConn1 -- H-Bridge/RConn4 -- Controlled Voltage Source/RConn2 -- Controlled Voltage Source4/RConn2 -- Controlled Voltage Source5/RConn2
  Revolute Joint/RConn2 -- PS-Simulink Converter/LConn1
  Ideal Angular Velocity Source1/RConn2 -- DC Motor1/RConn2 -- Mechanical Rotational Reference1/LConn1
  Ideal Angular Velocity Source1/LConn1 -- Ideal Torque Sensor1/RConn1
  Ideal Torque Sensor1/RConn2 -- Revolute Joint1/LConn2
  PS-Simulink Converter2/LConn1 -- Revolute Joint1/RConn2
  Ideal Angular Velocity Source1/RConn1 -- PS-Simulink Converter3/LConn1 -- Revolute Joint1/RConn3
  DC Motor1/LConn2 -- Simple Gear/LConn1
  Simple Gear/RConn1 -- Ideal Torque Sensor1/LConn1
  Rigid Transform5/RConn1 -- Revolute Joint1/LConn1
  Rigid Transform6/LConn1 -- Revolute Joint1/RConn1
  Rigid Transform6/RConn1 -- Rigid Transform2/LConn1
  PS-Simulink Converter5/LConn1 -- Prismatic Joint/RConn2
  Mechanical Translational Reference/LConn1 -- Ideal Translational Velocity Source/RConn2
  Ideal Translational Velocity Source/LConn1 -- Ideal Force Sensor/RConn1
  Ideal Translational Velocity Source/RConn1 -- Prismatic Joint/RConn3 -- PS-Simulink Converter4/LConn1
  Ideal Force Sensor/RConn2 -- Prismatic Joint/LConn2
  Ideal Force Sensor/LConn1 -- Leadscrew/RConn1
  DC Motor2/LConn2 -- Leadscrew/LConn1
  Mechanical Rotational Reference2/LConn1 -- DC Motor2/RConn2
  Prismatic Joint/RConn1 -- File Solid3/RConn1
  Prismatic Joint/LConn1 -- Rigid Transform4/RConn1
  H-Bridge/RConn2 -- Voltage Sensor/LConn1 -- DC Motor/LConn1
  H-Bridge/RConn3 -- Voltage Sensor/RConn2 -- DC Motor/RConn1
  H-Bridge/LConn1 -- Controlled Voltage Source/LConn1
  Simulink-PS Converter/RConn1 -- Controlled Voltage Source/RConn1
  Simulink-PS Converter2/RConn1 -- Controlled Voltage Source3/RConn1
  H-Bridge/LConn3 -- Controlled Voltage Source3/LConn1
  H-Bridge1/RConn1 -- Current Sensor/RConn2 -- H-Bridge2/RConn1 -- H-Bridge/RConn1
  PS-Simulink Converter7/LConn1 -- Voltage Sensor/RConn1
  DC Motor1/LConn1 -- Voltage Sensor1/LConn1 -- H-Bridge1/RConn2
  H-Bridge1/RConn3 -- Voltage Sensor1/RConn2 -- DC Motor1/RConn1
  Controlled Voltage Source5/LConn1 -- H-Bridge1/LConn1
  Controlled Voltage Source4/LConn1 -- H-Bridge1/LConn3
  Simulink-PS Converter4/RConn1 -- Controlled Voltage Source5/RConn1
  Simulink-PS Converter3/RConn1 -- Controlled Voltage Source4/RConn1
  DC Motor2/LConn1 -- Voltage Sensor2/LConn1 -- H-Bridge2/RConn2
  DC Motor2/RConn1 -- Voltage Sensor2/RConn2 -- H-Bridge2/RConn3
  Controlled Voltage Source1/LConn1 -- H-Bridge2/LConn1
  Controlled Voltage Source6/LConn1 -- H-Bridge2/LConn3
  Simulink-PS Converter6/RConn1 -- Controlled Voltage Source1/RConn1
  Simulink-PS Converter5/RConn1 -- Controlled Voltage Source6/RConn1
  DC Voltage Source/LConn1 -- Current Sensor/LConn1
  Current Sensor/RConn1 -- PS-Simulink Converter8/LConn1
  PS-Simulink Converter6/LConn1 -- Voltage Sensor1/RConn1
  PS-Simulink Converter9/LConn1 -- Voltage Sensor2/RConn1
